simulink model "chaine_base"  (R2023b)
settings: Solver=FixedStepDiscrete  StartTime=0.0  StopTime=Nb*Tb  FixedStep=Te  RelTol=1e-3
undefined symbols (not defined in the file): A, graine, L, psrc, seuil, sig2, Tb, Te
libraries: dspstat3 x1, simulink x1
settings Model: Creator=e2507457  LastModifiedBy=e2507457

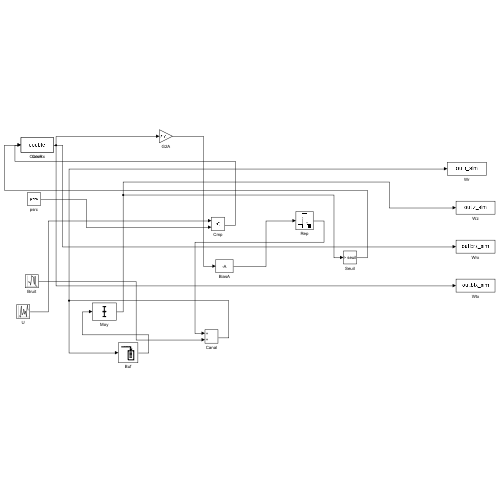
[thumbnail: Simulink's stored preview of the top-level diagram]
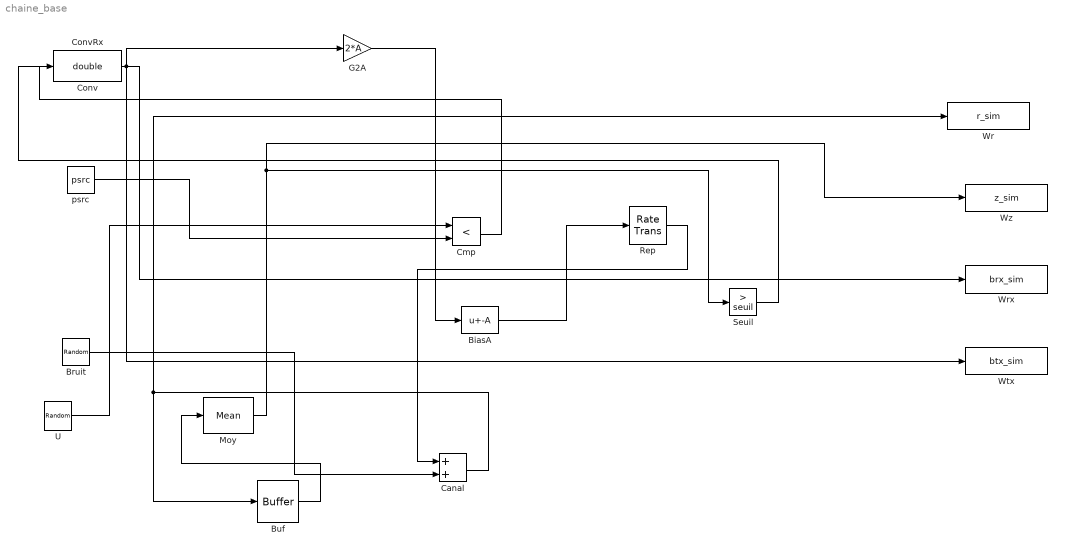
== system chaine_base ==
  BiasA : Bias  Bias=-A  SaturateOnIntegerOverflow=off
  Bruit : RandomNumber  Variance=sig2  Seed=graine+1  SampleTime=Te
  Buf : Buffer  N=L
  Canal : Sum
  Cmp : RelationalOperator  Operator=<  OutDataTypeStr=boolean  RndMeth=Simplest  InputSameDT=off
  Conv : DataTypeConversion  OutDataTypeStr=double  SaturateOnIntegerOverflow=off  RndMeth=Floor
  ConvRx : DataTypeConversion  OutDataTypeStr=double  SaturateOnIntegerOverflow=off  RndMeth=Floor
  G2A : Gain  Gain=2*A
  Moy : dspstat3/Mean  run=off  InputProcessing=Columns as channels (frame based)  reset_popup=None  directionMode=Each column  dimension=1  roiEnable=off  roiType=Rectangles  roiPortion=Entire ROI  roiOutput=Individual statistics for each ROI  roiFlag=off  roundingMode=Floor  overflowMode=off  outputDataTypeStr=Inherit: Same as accumulator  outputMin=[]  outputMax=[]  outputLastDataTypeStr=Inherit: Same as accumulator
  Rep : RateTransition  Integrity=off  Deterministic=off  OutPortSampleTime=Te
  Seuil : simulink/Logic and Bit Operations/Compare To Constant  relop=>  const=seuil  OutDataTypeStr=boolean
  U : UniformRandomNumber  Minimum=0  Seed=graine  SampleTime=Tb
  Wr : ToWorkspace  VariableName=r_sim  SampleTime=-1
  Wrx : ToWorkspace  VariableName=brx_sim  SampleTime=-1
  Wtx : ToWorkspace  VariableName=btx_sim  SampleTime=-1
  Wz : ToWorkspace  VariableName=z_sim  SampleTime=-1
  psrc : Constant  Value=psrc  SampleTime=Tb
  wires:
  U/1 -> Cmp/1
  psrc/1 -> Cmp/2
  Cmp/1 -> Conv/1
  Conv/1 -> G2A/1, Wtx/1
  G2A/1 -> BiasA/1
  BiasA/1 -> Rep/1
  Rep/1 -> Canal/1
  Bruit/1 -> Canal/2
  Canal/1 -> Wr/1, Buf/1
  Buf/1 -> Moy/1
  Moy/1 -> Wz/1, Seuil/1
  Seuil/1 -> ConvRx/1
  ConvRx/1 -> Wrx/1
